simulink model "Lab2_VM_Task_1234"  (R2018a)
settings: Solver=FixedStepDiscrete  StartTime=0.0  StopTime=Inf  FixedStep=0.02  RelTol=1e-3  EnableMultiTasking=on
undefined symbols (not defined in the file): Angular, Linear
libraries: robotlib x3
settings Model: Creator=The MathWorks, Inc.  LastModifiedBy=Sina
settings DataIOCC: LimitDataPoints=on  SaveFormat=Array
settings OptimizationCC: LifeSpan=Inf  MaxStackSize=64
settings DebuggingCC: SolverPrmCheckMsg=warning  AllowSymbolicDim=off  SFUnexpectedBacktrackingDiag=warning  SFNoUnconditionalDefaultTransitionDiag=warning  SFExecutionAtInitializationDiag=none
settings HardwareCC: ProdBitPerPointer=32  ProdBitPerSizeT=32  ProdBitPerPtrDiffT=32  ProdLargestAtomicFloat=None  ProdIntDivRoundTo=Undefined  ProdEndianess=Unspecified  ProdWordSize=32  ProdHWDeviceType=Generic->Unspecified (assume 32-bit Generic)  TargetHWDeviceType=Generic->Unspecified (assume 32-bit Generic)  UseEmbeddedCoderFeatures=off
settings ModelReferenceCC: PropagateSignalLabelsOutOfModel=off
settings RTWCC: SystemTargetFile=ert.tlc  HardwareBoard=Robot Operating System (ROS)  TemplateMakefile=ert_default_tmf  Toolchain=Catkin  TargetLang=C++
settings CodeAppCC: StateflowObjectComments=on
settings ERTTargetCC: MultiwordLength=2048  ERTCustomFileBanners=off  MultiInstanceERTCode=on  CodeInterfacePackaging=C++ class  SupportContinuousTime=on  SupportNonInlinedSFcns=on  RemoveResetFunc=off  SupportVariableSizeSignals=on  ModelStepFunctionPrototypeControlCompliant=off  RootIOFormat=Structure reference  ConvertIfToSwitch=off  SuppressUnreachableDefaultCases=off
settings ConfigComp: CovMetricSettings=dw  CovHtmlReporting=on  CovSaveCumulativeToWorkspaceVar=on  CovSaveSingleToWorkspaceVar=on  CovExternalEMLEnable=off  CovSFcnEnable=off

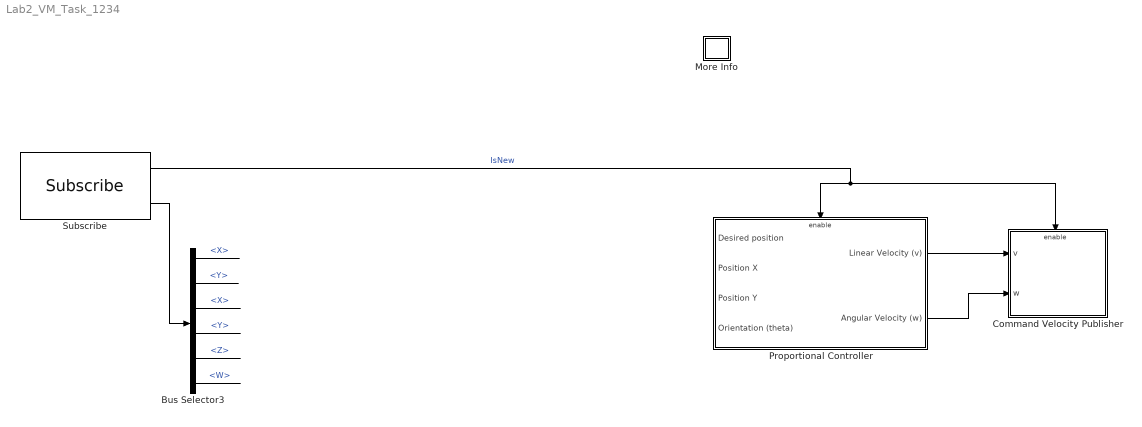
== system Lab2_VM_Task_1234 ==
  Bus Selector3 : BusSelector  OutputSignals=Pose.Pose.Position.X,Pose.Pose.Position.Y,Pose.Pose.Orientation.X,Pose.Pose.Orientation.Y,Pose.Pose.Orientation.Z,Pose.Pose.Orientation.W
  Command Velocity Publisher : Subsystem
  More Info : Subsystem
      settings: OpenFcn=showdemo(bdroot(gcb))
      mask Display: disp('?')
  Proportional Controller : Subsystem
  Subscribe : robotlib/Subscribe  SourceLibraryInfo=This block requires Robotics System Toolbox  topicSource=Select from ROS network  topic=/odom  messageType=nav_msgs/Odometry  sampleTime=-1  messageQueueLength=51
      settings: SourceProductBaseCode=RO
  wires:
  Subscribe/2 -> Bus Selector3/1
  Proportional Controller/1(Linear Velocity (v)) -> Command Velocity Publisher/1(v)
  Subscribe/1 -> Command Velocity Publisher/Enable, Proportional Controller/Enable  "IsNew"
  Bus Selector3/3 -> ?  "<X>"
  Bus Selector3/4 -> ?  "<Y>"
  Bus Selector3/5 -> ?  "<Z>"
  Bus Selector3/6 -> ?  "<W>"
  Proportional Controller/2(Angular Velocity (w)) -> Command Velocity Publisher/2(w)
  Bus Selector3/2 -> ?  "<Y>"
  Bus Selector3/1 -> ?  "<X>"

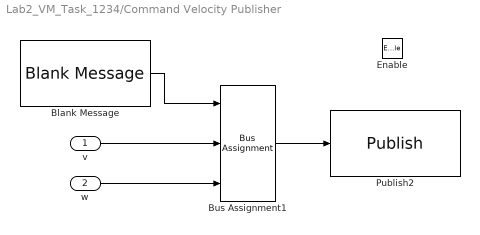
== system Lab2_VM_Task_1234/Command Velocity Publisher ==
  v : Inport
  w : Inport  Port=2
  Enable : EnablePort
  Blank Message : robotlib/Blank Message  SourceLibraryInfo=This block requires Robotics System Toolbox  messageType=geometry_msgs/Twist  SampleTime=inf
      settings: SourceProductBaseCode=RO
  Bus Assignment1 : BusAssignment  DialogController=Simulink.DDGSource_BusAssignment  AssignedSignals=Linear.X,Angular.Z
  Publish2 : robotlib/Publish  SourceLibraryInfo=This block requires Robotics System Toolbox  topicSource=Select from ROS network  topic=/cmd_vel  messageType=geometry_msgs/Twist  messageQueueLength=105
      settings: SourceProductBaseCode=RO
  wires:
  Bus Assignment1/1 -> Publish2/1
  Blank Message/1 -> Bus Assignment1/1
  v/1 -> Bus Assignment1/2
  w/1 -> Bus Assignment1/3

== system Lab2_VM_Task_1234/More Info ==

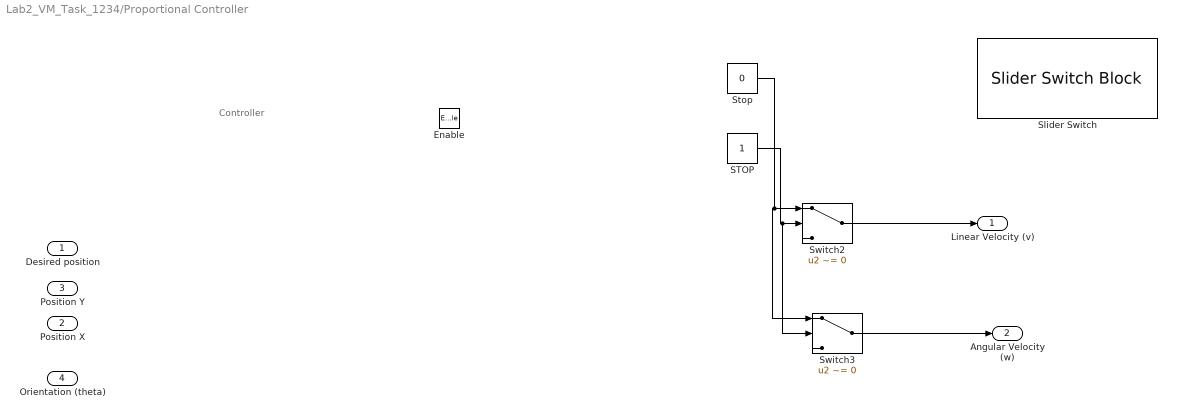
== system Lab2_VM_Task_1234/Proportional Controller ==
  note: Controller
  Desired position : Inport
  Position X : Inport  Port=2
  Position Y : Inport  Port=3
  Orientation (theta) : Inport  Port=4
  Enable : EnablePort
  "STOP " : Constant
  Slider Switch : SliderSwitchBlock  WebBlockId=158
      settings: Values={{'Off', 'On'}, [0 1]}
  Stop : Constant  Value=0
  Switch2 : Switch  Criteria=u2 ~= 0
  Switch3 : Switch  Criteria=u2 ~= 0
  Linear Velocity (v) : Outport
  Angular Velocity (w) : Outport  Port=2
  wires:
  Stop/1 -> Switch3/1, Switch2/1
  "STOP "/1 -> Switch3/2, Switch2/2
  Switch2/1 -> Linear Velocity (v)/1
  Switch3/1 -> Angular Velocity (w)/1
